simulink model "ElectricVehicleThermalManagementWithHeatPump_2026a_version"  (R2026a)
settings: Solver=VariableStepAuto  StopTime=3600  AbsTol=1e-3
PreLoadFcn:
  | init_nmpc
InitFcn:
  | init_nmpc
model workspace: external: MATLAB File ElectricVehicleThermalManagementWithHeatPumpParameters.m (data not in the file)
values from neighbouring files (symbols this model uses):
  battery_C1_LUT = [1913.6 12447 30609 ... (first row only)    [ElectricVehicleThermalManagementWithHeatPumpParameters.m]
  battery_capacity_LUT = [280.081 276.25 276.392]    [ElectricVehicleThermalManagementWithHeatPumpParameters.m]
  battery_cell_cp = 795    [ElectricVehicleThermalManagementWithHeatPumpParameters.m]
  battery_cell_mass = 2.5    [ElectricVehicleThermalManagementWithHeatPumpParameters.m]
  battery_Em_LUT = [3.4966 3.5057 3.5148 ... (first row only)    [ElectricVehicleThermalManagementWithHeatPumpParameters.m]
  battery_N_cells = 20    [ElectricVehicleThermalManagementWithHeatPumpParameters.m]
  battery_Qe_init = 0    [ElectricVehicleThermalManagementWithHeatPumpParameters.m]
  battery_R0_LUT = [0.0117 0.0085 0.009 ... (first row only)    [ElectricVehicleThermalManagementWithHeatPumpParameters.m]
  battery_R1_LUT = [0.0109 0.0029 0.0013 ... (first row only)    [ElectricVehicleThermalManagementWithHeatPumpParameters.m]
  battery_SOC_LUT = [0; 0.1; 0.25; 0.5; 0.75; 0.9; 1]    [ElectricVehicleThermalManagementWithHeatPumpParameters.m]
  battery_T_init = -5    [ElectricVehicleThermalManagementWithHeatPumpParameters.m]
  battery_temperature_LUT = [5 20 40]    [ElectricVehicleThermalManagementWithHeatPumpParameters.m]
  cabin_duct_area = 0.04    [ElectricVehicleThermalManagementWithHeatPumpParameters.m]
  cabin_T_init = -5    [ElectricVehicleThermalManagementWithHeatPumpParameters.m]
  chiller_area_primary = 0.43982297150257105    (= 0.439822971503)    [ElectricVehicleThermalManagementWithHeatPumpParameters.m]
  chiller_N_baffles = 3    [ElectricVehicleThermalManagementWithHeatPumpParameters.m]
  chiller_N_tubes = 100    [ElectricVehicleThermalManagementWithHeatPumpParameters.m]
  chiller_tube_D = 0.0035    [ElectricVehicleThermalManagementWithHeatPumpParameters.m]
  chiller_tube_L = 0.4    [ElectricVehicleThermalManagementWithHeatPumpParameters.m]
  chiller_wall_conductivity = 240    [ElectricVehicleThermalManagementWithHeatPumpParameters.m]
  chiller_wall_thickness = 0.0001    [ElectricVehicleThermalManagementWithHeatPumpParameters.m]
  cond_evap_air_area_flow = 0.3906    [ElectricVehicleThermalManagementWithHeatPumpParameters.m]
  cond_evap_air_area_primary = 1.4834999999999998    (= 1.4835)    [ElectricVehicleThermalManagementWithHeatPumpParameters.m]
  cond_evap_W = 0.015    [ElectricVehicleThermalManagementWithHeatPumpParameters.m]
  cond_evap_wall_conductivity = 240    [ElectricVehicleThermalManagementWithHeatPumpParameters.m]
  cond_evap_wall_thickness = 0.0001    [ElectricVehicleThermalManagementWithHeatPumpParameters.m]
  coolant_channel_D = 0.0092    [ElectricVehicleThermalManagementWithHeatPumpParameters.m]
  coolant_pipe_D = 0.019    [ElectricVehicleThermalManagementWithHeatPumpParameters.m]
  coolant_T_init = -5    [ElectricVehicleThermalManagementWithHeatPumpParameters.m]
  coolant_tank_area = 0.0121    [ElectricVehicleThermalManagementWithHeatPumpParameters.m]
  coolant_tank_volume = 1.25    [ElectricVehicleThermalManagementWithHeatPumpParameters.m]
  coolant_valve_D_ratio_max = 0.95    [ElectricVehicleThermalManagementWithHeatPumpParameters.m]
  coolant_valve_D_ratio_min = 0.001    [ElectricVehicleThermalManagementWithHeatPumpParameters.m]
  coolant_valve_displacement = 0.0063    [ElectricVehicleThermalManagementWithHeatPumpParameters.m]
  coolant_valve_S_max = 0.0053    [ElectricVehicleThermalManagementWithHeatPumpParameters.m]
  evaporator_air_area_flow = 0.12    [ElectricVehicleThermalManagementWithHeatPumpParameters.m]
  evaporator_air_area_primary = 0.4323    [ElectricVehicleThermalManagementWithHeatPumpParameters.m]
  evaporator_W = 0.015    [ElectricVehicleThermalManagementWithHeatPumpParameters.m]
  evaporator_wall_conductivity = 240    [ElectricVehicleThermalManagementWithHeatPumpParameters.m]
  evaporator_wall_thickness = 0.0001    [ElectricVehicleThermalManagementWithHeatPumpParameters.m]
  expansion_valve_D_ratio_max = 0.9    [ElectricVehicleThermalManagementWithHeatPumpParameters.m]
  hex_area_primary = 0.070371675440411369    (= 0.0703716754404)    [ElectricVehicleThermalManagementWithHeatPumpParameters.m]
  hex_N_tubes = 64    [ElectricVehicleThermalManagementWithHeatPumpParameters.m]
  hex_tube_D = 0.0035    [ElectricVehicleThermalManagementWithHeatPumpParameters.m]
  hex_wall_conductivity = 240    [ElectricVehicleThermalManagementWithHeatPumpParameters.m]
  hex_wall_thickness = 0.0001    [ElectricVehicleThermalManagementWithHeatPumpParameters.m]
  inner_cond_air_area_flow = 0.1953    [ElectricVehicleThermalManagementWithHeatPumpParameters.m]
  inner_cond_air_area_primary = 0.99520000000000008    (= 0.9952)    [ElectricVehicleThermalManagementWithHeatPumpParameters.m]
  inner_cond_W = 0.02    [ElectricVehicleThermalManagementWithHeatPumpParameters.m]
  inner_cond_wall_conductivity = 240    [ElectricVehicleThermalManagementWithHeatPumpParameters.m]
  inner_cond_wall_thickness = 0.0001    [ElectricVehicleThermalManagementWithHeatPumpParameters.m]
  pump_speed_max = 1000    [ElectricVehicleThermalManagementWithHeatPumpParameters.m]
  radiator_air_area_flow = 0.097499999999999989    (= 0.0975)    [ElectricVehicleThermalManagementWithHeatPumpParameters.m]
  radiator_air_area_primary = 0.43687499999999996    (= 0.436875)    [ElectricVehicleThermalManagementWithHeatPumpParameters.m]
  radiator_W = 0.015    [ElectricVehicleThermalManagementWithHeatPumpParameters.m]
  radiator_wall_conductivity = 240    [ElectricVehicleThermalManagementWithHeatPumpParameters.m]
  radiator_wall_thickness = 0.0001    [ElectricVehicleThermalManagementWithHeatPumpParameters.m]
  refrigerant_p_init = 0.25    [ElectricVehicleThermalManagementWithHeatPumpParameters.m]
  refrigerant_pipe_D = 0.01    [ElectricVehicleThermalManagementWithHeatPumpParameters.m]
  refrigerant_valve_D_ratio_max = 0.95    [ElectricVehicleThermalManagementWithHeatPumpParameters.m]
  refrigerant_valve_displacement = 0.005    [ElectricVehicleThermalManagementWithHeatPumpParameters.m]
libraries: fl_lib x227, nesl_utility x162, SimscapeFluids_lib x30, LiBatteryElements_lib x16, slpidlib x3, SignalEditorBlockLib x1
(part 3 of 13)

== system ElectricVehicleThermalManagementWithHeatPump_2026a_version/Chiller ==
  Chiller : SimscapeFluids_lib/Heat Exchangers/Two-Phase Fluid - Thermal Liquid/Condenser Evaporator (TL-2P)  flow_arrangement=fluids.heat_exchangers.enum.FlowArrangementTL2P.Cross  cross_flow_arrangement=fluids.heat_exchangers.enum.CrossFlowArrangementTL2P.UnmixedMixed  R_wall=chiller_wall_thickness / chiller_area_primary / chiller_wall_conductivity K/W  wall_thermal_mass=false  mass_wall=1 kg  cp_wall=490 J/(K*kg)  area_A1=pi * coolant_pipe_D^2 / 4 m^2  area_B1=pi * coolant_pipe_D^2 / 4 m^2  area_A2=pi * refrigerant_pipe_D^2 / 4 m^2  area_B2=pi * refrigerant_pipe_D^2 / 4 m^2  flow_geometry_TL=fluids.heat_exchangers.enum.FlowGeometryTL.AcrossTubeBank  tube_num_TL=1  tube_length_TL=5 m  tube_cross_section_TL=fluids.heat_exchangers.enum.TubeCrossSection.Circular  tube_diameter_TL=0.1 m  tube_width_TL=0.1 m  tube_height_TL=0.1 m  tube_inner_diameter_TL=0.05 m  tube_outer_diameter_TL=0.1 m  tube_flow_area_TL=0.01 m^2  tube_wetted_perimeter_TL=0.4 m  tube_heat_perimeter_TL=0.4 m  tube_pressure_loss_spec_TL=fluids.heat_exchangers.enum.TubePressureLossSpec.Haaland  tube_loss_coeff_TL=10  tube_local_pressure_loss_spec_TL=fluids.heat_exchangers.enum.LocalLossSpec.AggregateLength  tube_length_add_TL=0.1 m  tube_local_loss_coefficient_TL=0.1  tube_roughness_pressure_TL=15e-6 m  tube_Re_lam_pressure_TL=2000  tube_Re_tur_pressure_TL=4000  tube_shape_factor_generic_TL=64  tube_heat_coeff_spec_TL=fluids.heat_exchangers.enum.TubeHeatCoeffSpec.Gneilinski  tube_colburn_coeff_TL=[.023, .8, .33]  tube_roughness_heat_TL=15e-6 m  tube_Re_lam_heat_TL=2000  tube_Re_tur_heat_TL=4000  tube_Nu_lam_generic_TL=3.66  bank_arrangement_TL=fluids.heat_exchangers.enum.BankArrangement.Staggered  bank_num_rows_TL=sqrt(chiller_N_tubes) * (chiller_N_baffles + 1)  bank_tubes_per_row_TL=sqrt(chiller_N_tubes)  bank_width_TL=chiller_tube_L / (chiller_N_baffles + 1) m  bank_tube_diameter_TL=chiller_tube_D m  bank_longitudinal_pitch_TL=2 * chiller_tube_D m  bank_transverse_pitch_TL=2 * chiller_tube_D m  bank_pressure_loss_spec_TL=fluids.heat_exchangers.enum.BankPressureLossSpec.Martin  bank_euler_TL=10  bank_heat_coeff_spec_TL=fluids.heat_exchangers.enum.BankHeatCoeffSpec.Martin  bank_colburn_coeff_TL=[.27, .63, .36]  generic_flow_area_TL=0.01 m^2  generic_heat_area_TL=2 m^2  generic_volume_TL=0.05 m^3  generic_loss_coeff_TL=10  generic_colburn_coeff_TL=[.023, .8, .33]  fouling_factor_TL=0.1 m^2*K/kW  fin_area_TL=chiller_area_baffles m^2  fin_efficiency_TL=0.5  p_init_TL=coolant_p_init MPa  T_init_TL=coolant_T_init degC  tube_num_2P=chiller_N_tubes  tube_length_2P=chiller_tube_L m  tube_cross_section_2P=fluids.heat_exchangers.enum.TubeCrossSection.Circular  tube_diameter_2P=chiller_tube_D m  tube_width_2P=0.1 m  tube_height_2P=0.1 m  tube_inner_diameter_2P=0.05 m  tube_outer_diameter_2P=0.1 m  tube_flow_area_2P=0.01 m^2  tube_wetted_perimeter_2P=0.4 m  tube_heat_perimeter_2P=0.4 m  tube_pressure_loss_spec_2P=fluids.heat_exchangers.enum.TubePressureLossSpec2P.Haaland  tube_loss_coeff_2P=10  tube_local_pressure_loss_spec_2P=fluids.heat_exchangers.enum.LocalLossSpec.AggregateLength  tube_length_add_2P=chiller_tube_Leq m  tube_local_loss_coefficient_2P=0.1  tube_roughness_pressure_2P=15e-6 m  tube_Re_lam_pressure_2P=2000  tube_Re_tur_pressure_2P=4000  tube_shape_factor_generic_2P=64  tube_heat_coeff_spec_2P=fluids.heat_exchangers.enum.TubeHeatCoeffSpec2P.GneilinskiCavalliniZecchin  tube_colburn_coeff_liq_2P=[.023, .8, .33]  tube_colburn_coeff_mix_2P=[.05, .8, .33]  tube_colburn_coeff_vap_2P=[.023, .8, .33]  tube_roughness_heat_2P=15e-6 m  tube_Re_lam_heat_2P=2000  tube_Re_tur_heat_2P=4000  tube_Nu_lam_generic_2P=3.66  fouling_factor_2P=0.1 m^2*K/kW  fin_area_2P=0 m^2  fin_efficiency_2P=0  energy_spec_2P=foundation.enum.energy_spec.void_fraction  p_init_2P=refrigerant_p_init MPa  T_init_2P=293.15 K  x_init_2P=0.5  alpha_init_2P=refrigerant_alpha_init  h_init_2P=1500 kJ/kg  u_init_2P=1500 kJ/kg
  Flow Resistance (2P) : fl_lib/Two-Phase Fluid/Elements/Flow Resistance (2P)  delta_p_nominal=1e-4 MPa  mdot_nominal=0.01 kg/s  v_nominal=0 m^3/kg  area=pi * refrigerant_pipe_D^2 / 4 m^2  laminar_fraction=1e-3
  PS-Simulink Converter : nesl_utility/PS-Simulink Converter  PhysicalDomain=network_engine_domain  SubClassName=ps_output  LeftPortType=input  RightPortType=output  PseudoPeriodic=off  Frequencies=[]  VectorFormat=inherit  Unit=inherit  AffineConversion=off
  PS-Simulink Converter1 : nesl_utility/PS-Simulink Converter  PhysicalDomain=network_engine_domain  SubClassName=ps_output  LeftPortType=input  RightPortType=output  PseudoPeriodic=off  Frequencies=[]  VectorFormat=inherit  Unit=inherit  AffineConversion=off
  Pressure & Temperature Sensor (TL) : fl_lib/Thermal Liquid/Sensors/Pressure & Temperature Sensor (TL)  reference=foundation.enum.MeasurementReference.absolute  pressure=true  pressure_spec=foundation.enum.PressureMeasementSpec.Absolute  temperature=true
  Pressure & Temperature Sensor (TL)1 : fl_lib/Thermal Liquid/Sensors/Pressure & Temperature Sensor (TL)  reference=foundation.enum.MeasurementReference.absolute  pressure=true  pressure_spec=foundation.enum.PressureMeasementSpec.Absolute  temperature=true
  SR10 : Subsystem
  SR9 : Subsystem
  To Workspace : ToWorkspace  VariableName=clntChilTemp_in  SampleTime=-1
  To Workspace1 : ToWorkspace  VariableName=clntChilTemp_out  SampleTime=-1
  C : PMIOPort  Side=Left
  A : PMIOPort  Port=2  Side=Left
  D : PMIOPort  Port=3  Side=Right
  B : PMIOPort  Port=4  Side=Right
  wires:
  PS-Simulink Converter/1 -> To Workspace/1
  PS-Simulink Converter1/1 -> To Workspace1/1
  connections:
  SR10/LConn1 -- Chiller/RConn2
  SR10/RConn1 -- Flow Resistance (2P)/LConn1
  B/RConn1 -- Flow Resistance (2P)/RConn1
  SR9/RConn1 -- Chiller/RConn1
  Chiller/LConn2 -- Pressure & Temperature Sensor (TL)1/LConn1 -- D/RConn1
  Chiller/LConn1 -- Pressure & Temperature Sensor (TL)/LConn1 -- C/RConn1
  SR9/LConn1 -- A/RConn1
  PS-Simulink Converter/LConn1 -- Pressure & Temperature Sensor (TL)/RConn2
  PS-Simulink Converter1/LConn1 -- Pressure & Temperature Sensor (TL)1/RConn2

== system ElectricVehicleThermalManagementWithHeatPump_2026a_version/Chiller Expansion Valve ==
  Chiller Expansion Valve : SimscapeFluids_lib/Two-Phase Fluid/Valves & Orifices/Orifice (2P)  orifice_type=foundation.enum.constant_variable.variable  constant_liquid_orifice_parameterization=fluids.two_phase_fluid.valves_orifices.enum.LiquidConstantOrificeParameterization.Area  variable_liquid_orifice_parameterization=fluids.two_phase_fluid.valves_orifices.enum.LiquidOrificeParameterization.LinearArea  mdot_nominal_constant=0.1 kg/s  delta_p_nominal_constant=0.001 MPa  orifice_area_constant=1e-4 m^2  S_min=0 m  del_S=refrigerant_valve_displacement m  open_orientation=fluids.two_phase_fluid.valves_orifices.enum.OrificeOrientation.Positive  mdot_nominal_max=0.1 kg/s  delta_p_nominal_max=0.001 MPa  orifice_area_max=pi * (expansion_valve_D_ratio_max*refrigerant_pipe_D)^2 / 4 m^2  S_TLU=[0, .002, .004, .007, .017] m  orifice_area_TLU=[1e-10, 2e-05, 4e-05, 6e-05, 8e-05, .0001] m^2  energy_spec=foundation.enum.energy_spec.temperature  p_inlet=0.101325 MPa  T_inlet=293.15 K  x_inlet=0  alpha_inlet=0  h_inlet=400 kJ/kg  u_inlet=400 kJ/kg  Cd=0.7  pressure_recovery=true  leakage_fraction=1e-6  smoothing_factor=0.01  B_lam=0.999  tau_x=0.1 s  area=pi * refrigerant_pipe_D^2 / 4 m^2  vapor_orifice_parameterization=fluids.two_phase_fluid.valves_orifices.enum.VaporOrificeParameterization.Cv  opening_characteristic=fluids.two_phase_fluid.valves_orifices.enum.OpeningCharacteristics.Linear  Cv_constant=4  Cv_max=4  S_Cv_TLU=[0, .003, .006, .009, .012, .015] m  Cv_TLU=[1e-06, .8, 1.6, 2.4, 3.2, 4]  xT_Cv=0.7  Kv_constant=3.6  Kv_max=3.6  S_Kv_TLU=[0, .003, .006, .009, .012, .015] m  Kv_TLU=[1e-06, .72, 1.44, 2.16, 2.88, 3.6]  xT_Kv=0.7  S_orifice_area_TLU=[0, .003, .006, .009, .012, .015] m
  Display : Display
  Max Valve Displacement [m] : Gain  Gain=refrigerant_valve_displacement
  Scope : Scope
      settings: ActiveDisplayYMinimum=-0.003  ActiveDisplayYMaximum=0.027  DataLoggingVariableName=ScopeData3
  Scope1 : Scope
      settings: ActiveDisplayYMinimum=-0.003  ActiveDisplayYMaximum=0.027  DataLoggingVariableName=ScopeData4
  Scope2 : Scope
      settings: ActiveDisplayYMinimum=-1E-5  ActiveDisplayYMaximum=0.00014  DataLoggingVariableName=ScopeData5
  Simulink-PS Converter : nesl_utility/Simulink-PS Converter  PhysicalDomain=network_engine_domain  SubClassName=ps_input  LeftPortType=input  RightPortType=output  PseudoPeriodic=off  Frequencies=[]  NoiseDistribution=none  NoiseParameters=[]  Unit=m  AffineConversion=off  FilteringAndDerivatives=provide  SimscapeFilterOrder=1  InputFilterTimeConstant=0.001  UdotUserProvided=0
  Transfer Fcn : TransferFcn  Denominator=[1 1]
  A : PMIOPort  Side=Left
  B : PMIOPort  Port=2  Side=Right
  wires:
  Max Valve Displacement [m]/1 -> Display/1, Scope2/1, Simulink-PS Converter/1
  [cmd_exv_chiller] -> Scope1/1, Transfer Fcn/1
  Transfer Fcn/1 -> Scope/1, Max Valve Displacement [m]/1
  connections:
  Chiller Expansion Valve/RConn1 -- B/RConn1
  Chiller Expansion Valve/LConn1 -- A/RConn1
  Chiller Expansion Valve/LConn2 -- Simulink-PS Converter/RConn1

== system ElectricVehicleThermalManagementWithHeatPump_2026a_version/Chiller Evaporator Bypass Valve ==
  Bias : Bias  Bias=-1  SaturateOnIntegerOverflow=off
  Gain : Gain  Gain=2
  Max Valve Displacement [m] : Gain  Gain=refrigerant_valve_displacement
  Orifice AB : SimscapeFluids_lib/Two-Phase Fluid/Valves & Orifices/Orifice (2P)  orifice_type=foundation.enum.constant_variable.variable  constant_liquid_orifice_parameterization=fluids.two_phase_fluid.valves_orifices.enum.LiquidConstantOrificeParameterization.Area  variable_liquid_orifice_parameterization=fluids.two_phase_fluid.valves_orifices.enum.LiquidOrificeParameterization.LinearArea  mdot_nominal_constant=0.1 kg/s  delta_p_nominal_constant=0.001 MPa  orifice_area_constant=1e-4 m^2  S_min=-0.8*refrigerant_valve_displacement m  del_S=refrigerant_valve_displacement m  open_orientation=fluids.two_phase_fluid.valves_orifices.enum.OrificeOrientation.Positive  mdot_nominal_max=0.1 kg/s  delta_p_nominal_max=0.001 MPa  orifice_area_max=pi * (refrigerant_valve_D_ratio_max*refrigerant_pipe_D)^2 / 4 m^2  S_TLU=[0, .002, .004, .007, .017] m  orifice_area_TLU=[1e-10, 2e-05, 4e-05, 6e-05, 8e-05, .0001] m^2  energy_spec=foundation.enum.energy_spec.temperature  p_inlet=0.101325 MPa  T_inlet=293.15 K  x_inlet=0  alpha_inlet=0  h_inlet=400 kJ/kg  u_inlet=400 kJ/kg  Cd=0.7  pressure_recovery=true  leakage_fraction=1e-6  smoothing_factor=0.01  B_lam=0.999  tau_x=0.1 s  area=pi * refrigerant_pipe_D^2 / 4 m^2  vapor_orifice_parameterization=fluids.two_phase_fluid.valves_orifices.enum.VaporOrificeParameterization.Cv  opening_characteristic=fluids.two_phase_fluid.valves_orifices.enum.OpeningCharacteristics.Linear  Cv_constant=4  Cv_max=4  S_Cv_TLU=[0, .003, .006, .009, .012, .015] m  Cv_TLU=[1e-06, .8, 1.6, 2.4, 3.2, 4]  xT_Cv=0.7  Kv_constant=3.6  Kv_max=3.6  S_Kv_TLU=[0, .003, .006, .009, .012, .015] m  Kv_TLU=[1e-06, .72, 1.44, 2.16, 2.88, 3.6]  xT_Kv=0.7  S_orifice_area_TLU=[0, .003, .006, .009, .012, .015] m
  Orifice AC : SimscapeFluids_lib/Two-Phase Fluid/Valves & Orifices/Orifice (2P)  orifice_type=foundation.enum.constant_variable.variable  constant_liquid_orifice_parameterization=fluids.two_phase_fluid.valves_orifices.enum.LiquidConstantOrificeParameterization.Area  variable_liquid_orifice_parameterization=fluids.two_phase_fluid.valves_orifices.enum.LiquidOrificeParameterization.LinearArea  mdot_nominal_constant=0.1 kg/s  delta_p_nominal_constant=0.001 MPa  orifice_area_constant=1e-4 m^2  S_min=0.8*refrigerant_valve_displacement m  del_S=refrigerant_valve_displacement m  open_orientation=fluids.two_phase_fluid.valves_orifices.enum.OrificeOrientation.Negative  mdot_nominal_max=0.1 kg/s  delta_p_nominal_max=0.001 MPa  orifice_area_max=pi * (refrigerant_valve_D_ratio_max*refrigerant_pipe_D)^2 / 4 m^2  S_TLU=[0, .002, .004, .007, .017] m  orifice_area_TLU=[1e-10, 2e-05, 4e-05, 6e-05, 8e-05, .0001] m^2  energy_spec=foundation.enum.energy_spec.temperature  p_inlet=0.101325 MPa  T_inlet=293.15 K  x_inlet=0  alpha_inlet=0  h_inlet=400 kJ/kg  u_inlet=400 kJ/kg  Cd=0.7  pressure_recovery=true  leakage_fraction=1e-6  smoothing_factor=0.01  B_lam=0.999  tau_x=0.1 s  area=pi * refrigerant_pipe_D^2 / 4 m^2  vapor_orifice_parameterization=fluids.two_phase_fluid.valves_orifices.enum.VaporOrificeParameterization.Cv  opening_characteristic=fluids.two_phase_fluid.valves_orifices.enum.OpeningCharacteristics.Linear  Cv_constant=4  Cv_max=4  S_Cv_TLU=[0, .003, .006, .009, .012, .015] m  Cv_TLU=[1e-06, .8, 1.6, 2.4, 3.2, 4]  xT_Cv=0.7  Kv_constant=3.6  Kv_max=3.6  S_Kv_TLU=[0, .003, .006, .009, .012, .015] m  Kv_TLU=[1e-06, .72, 1.44, 2.16, 2.88, 3.6]  xT_Kv=0.7  S_orifice_area_TLU=[0, .003, .006, .009, .012, .015] m
  Scope : Scope
      settings: ActiveDisplayYMinimum=-1  ActiveDisplayYMaximum=1  DataLoggingVariableName=ScopeData2
  Simulink-PS Converter : nesl_utility/Simulink-PS Converter  PhysicalDomain=network_engine_domain  SubClassName=ps_input  LeftPortType=input  RightPortType=output  PseudoPeriodic=off  Frequencies=[]  NoiseDistribution=none  NoiseParameters=[]  Unit=m  AffineConversion=off  FilteringAndDerivatives=provide  SimscapeFilterOrder=1  InputFilterTimeConstant=0.001  UdotUserProvided=0
  Transfer Fcn : TransferFcn  Denominator=[1 1]
  C : PMIOPort  Side=Left
  A : PMIOPort  Port=2  Side=Right
  B : PMIOPort  Port=3  Side=Right
  wires:
  Transfer Fcn/1 -> Gain/1
  Bias/1 -> Max Valve Displacement [m]/1
  [cmd_refrig_bypass] -> Scope/1, Transfer Fcn/1
  Max Valve Displacement [m]/1 -> Simulink-PS Converter/1
  Gain/1 -> Bias/1
  connections:
  A/RConn1 -- Orifice AB/LConn1 -- Orifice AC/LConn1
  Orifice AC/RConn1 -- C/RConn1
  Orifice AB/RConn1 -- B/RConn1
  Simulink-PS Converter/RConn1 -- Orifice AB/LConn2 -- Orifice AC/LConn2

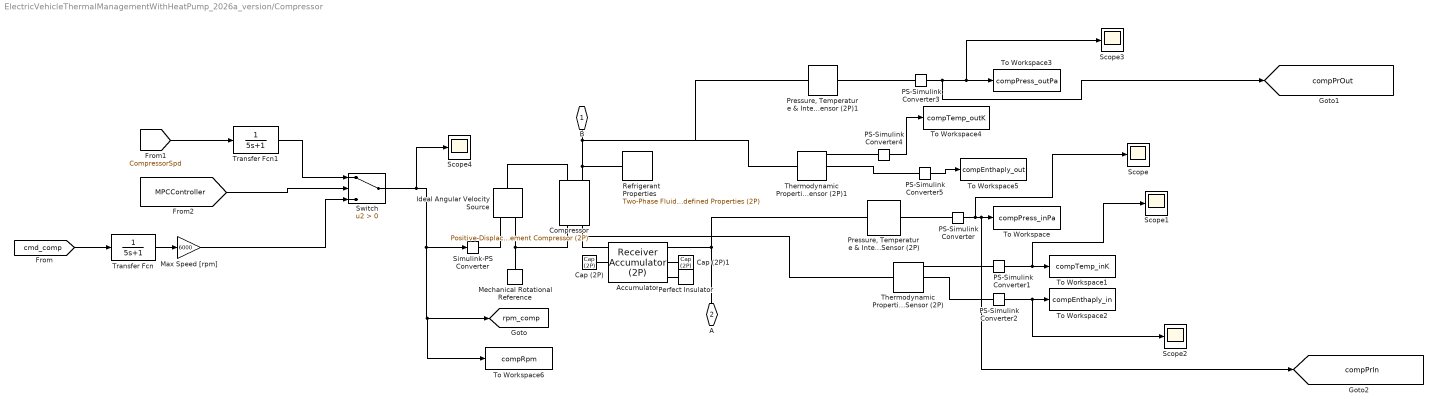
== system ElectricVehicleThermalManagementWithHeatPump_2026a_version/Compressor ==
  Accumulator : SimscapeFluids_lib/Two-Phase Fluid/Tanks & Accumulators/Receiver Accumulator (2P)  volume=4 l  tank_area=0.5 m^2  area_AV=pi * refrigerant_pipe_D^2 / 4 m^2  area_BV=pi * refrigerant_pipe_D^2 / 4 m^2  area_AL=pi * refrigerant_pipe_D^2 / 4 m^2  area_BL=pi * refrigerant_pipe_D^2 / 4 m^2  V_frac_liq_error=simscape.enum.assert.action.none  V_frac_liq_min=0.05  V_frac_liq_max=0.95  V_frac_smooth=0.05  p_crit_error=simscape.enum.assert.action.error  hc_vap=20 W/(K*m^2)  hc_liq=100 W/(K*m^2)  p_init=refrigerant_p_init MPa  fraction_spec=fluids.two_phase_fluid.tanks_accumulators.enum.LiquidFractionSpec.Volume  M_frac_liq_init=0.5  V_frac_liq_init=0.1  saturated_init=true  energy_spec=fluids.two_phase_fluid.tanks_accumulators.enum.EnergySpec.SubcoolingSuperheating  delta_T_sub_init=5 deltaK  delta_T_sup_init=5 deltaK  T_liq_init=368.15 K  T_vap_init=378.15 K  h_liq_init=400 kJ/kg  h_vap_init=2700 kJ/kg  u_liq_init=400 kJ/kg  u_vap_init=2700 kJ/kg  tau_vap_cond=0.1 s
  Cap (2P) : fl_lib/Two-Phase Fluid/Elements/Cap (2P)  p_specify=off  p_priority=None  p=0.101325 MPa  p_nominal_specify=off  p_nominal_value=1  p_nominal_unit=MPa  u_specify=off  u_priority=None  u=1500 kJ/kg  u_nominal_specify=off  u_nominal_value=1  u_nominal_unit=kJ/kg
  Cap (2P)1 : fl_lib/Two-Phase Fluid/Elements/Cap (2P)  p_specify=off  p_priority=None  p=0.101325 MPa  p_nominal_specify=off  p_nominal_value=1  p_nominal_unit=MPa  u_specify=off  u_priority=None  u=1500 kJ/kg  u_nominal_specify=off  u_nominal_value=1  u_nominal_unit=kJ/kg
  Compressor : SimscapeFluids_lib/Two-Phase Fluid/Fluid Machines/Positive-Displacement Compressor (2P)  dispSpec=fluids.two_phase_fluid.fluid_machines.enum.DisplacementSpecification.Displacement  v_disp=compressor_displacement cm^3/rev  mdot_nom=0.01 kg/s  omega_nom=1000 rpm  efficiencySpec=fluids.two_phase_fluid.fluid_machines.enum.VolumetricEfficiencyParameterization.Analytical  thermodynamicModelSpec=fluids.two_phase_fluid.fluid_machines.enum.ThermodynamicModel.Isentropic  n=1.2  eta_isen=0.65  eta_isen_TLU=[.95, .9, .85, .8, .75; .925, .875, .825, .775, .725; .875, .825, .775, .725, .675; .75, .7, .65, .6, .55]  eta_vol_nom=0.9  pr_TLU=[2, 4, 6, 8]  omega_TLU=[800, 1500, 2800, 3300, 4000] rpm  eta_vol_TLU=[.95, .9, .85, .8, .75; .925, .875, .825, .775, .725; .875, .825, .775, .725, .675; .75, .7, .65, .6, .55]  nominalSpec=fluids.two_phase_fluid.fluid_machines.enum.NominalConditionsSpecification.Pressure  pr_nom=4.6  p_in_nom=0.3 MPa  T_in_nom=11 degC  T_evap_nom=373.15 K  T_cond_nom=398.15 K  delta_T_nom=10 deltaK  mechanical_efficiency=0.95  area_A=pi * refrigerant_pipe_D^2 / 4 m^2  area_B=pi * refrigerant_pipe_D^2 / 4 m^2  VaporCheck=simscape.enum.assert.action.none
  Ideal Angular Velocity Source : fl_lib/Mechanical/Mechanical Sources/Ideal Angular Velocity Source
  Max Speed [rpm] : Gain  Gain=6000
  Mechanical Rotational Reference : fl_lib/Mechanical/Rotational Elements/Mechanical Rotational Reference
  PS-Simulink Converter{,1..5} (6 alike) : nesl_utility/PS-Simulink Converter  PhysicalDomain=network_engine_domain  SubClassName=ps_output  LeftPortType=input  RightPortType=output  PseudoPeriodic=off  Frequencies=[]  VectorFormat=inherit  Unit=inherit  AffineConversion=off
  Perfect Insulator : fl_lib/Thermal/Thermal Elements/Perfect Insulator  T_specify=off  T_priority=None  T=293.15 K  T_nominal_specify=off  T_nominal_value=1  T_nominal_unit=K
  "Pressure, Temperature & Internal Energy Sensor (2P)" : fl_lib/Two-Phase Fluid/Sensors/Pressure, Temperature & Internal Energy Sensor (2P)  reference=foundation.enum.MeasurementReference.absolute  pressure=true  pressure_spec=foundation.enum.PressureMeasementSpec.Absolute  temperature=false  internal_energy=false
  "Pressure, Temperature & Internal Energy Sensor (2P)1" : fl_lib/Two-Phase Fluid/Sensors/Pressure, Temperature & Internal Energy Sensor (2P)  reference=foundation.enum.MeasurementReference.absolute  pressure=true  pressure_spec=foundation.enum.PressureMeasementSpec.Absolute  temperature=false  internal_energy=false
  Refrigerant Properties : SimscapeFluids_lib/Two-Phase Fluid/Utilities/Two-Phase Fluid Predefined Properties (2P)  fluid=fluids.two_phase_fluid.utilities.enum.Fluid.R134a  p_atm=0.101325 MPa  properties_range_check=simscape.enum.assert.action.error  q_rev=0.01 Pa
  Scope{,1..4} (5 alike) : Scope
      Scope settings: ActiveDisplayYMinimum=0.05986  ActiveDisplayYMaximum=0.28314  DataLoggingVariableName=ScopeData10
      Scope1 settings: ActiveDisplayYMinimum=241.45357  ActiveDisplayYMaximum=273.1745  DataLoggingVariableName=ScopeData11
      Scope2 settings: ActiveDisplayYMinimum=334.35031  ActiveDisplayYMaximum=407.78163  DataLoggingVariableName=ScopeData12
      Scope3 settings: ActiveDisplayYMinimum=-0.28873  ActiveDisplayYMaximum=4.5986
      Scope4 settings: ActiveDisplayYMinimum=-746.11242  ActiveDisplayYMaximum=6715.0118  DataLoggingVariableName=ScopeData4
  Simulink-PS Converter : nesl_utility/Simulink-PS Converter  PhysicalDomain=network_engine_domain  SubClassName=ps_input  LeftPortType=input  RightPortType=output  PseudoPeriodic=off  Frequencies=[]  NoiseDistribution=none  NoiseParameters=[]  Unit=rpm  AffineConversion=off  FilteringAndDerivatives=provide  SimscapeFilterOrder=1  InputFilterTimeConstant=0.001  UdotUserProvided=0
  Switch : Switch  Criteria=u2 > Threshold  SaturateOnIntegerOverflow=off  InputSameDT=off
  Thermodynamic Properties Sensor (2P) : fl_lib/Two-Phase Fluid/Sensors/Thermodynamic Properties Sensor (2P)  temperature=true  enthalpy=true  density=true  specific_volume=false  entropy=false
  Thermodynamic Properties Sensor (2P)1 : fl_lib/Two-Phase Fluid/Sensors/Thermodynamic Properties Sensor (2P)  temperature=true  enthalpy=true  density=true  specific_volume=false  entropy=false
  To Workspace : ToWorkspace  VariableName=compPress_inPa  SampleTime=-1
  To Workspace1 : ToWorkspace  VariableName=compTemp_inK  SampleTime=-1
  To Workspace2 : ToWorkspace  VariableName=compEnthaply_in  SampleTime=-1
  To Workspace3 : ToWorkspace  VariableName=compPress_outPa  SampleTime=-1
  To Workspace4 : ToWorkspace  VariableName=compTemp_outK  SampleTime=-1
  To Workspace5 : ToWorkspace  VariableName=compEnthaply_out  SampleTime=-1
  To Workspace6 : ToWorkspace  VariableName=compRpm  SampleTime=-1
  Transfer Fcn : TransferFcn  Denominator=[5 1]
  Transfer Fcn1 : TransferFcn  Denominator=[5 1]
  B : PMIOPort  Side=Left
  A : PMIOPort  Port=2  Side=Right
  tag scope: compPrIn=global, compPrOut=global, rpm_comp=global
  wires:
  Transfer Fcn/1 -> Max Speed [rpm]/1
  [cmd_comp] -> Transfer Fcn/1
  Max Speed [rpm]/1 -> Switch/3
  PS-Simulink Converter/1 -> Scope/1, [compPrIn], To Workspace/1
  PS-Simulink Converter1/1 -> Scope1/1, To Workspace1/1
  PS-Simulink Converter2/1 -> Scope2/1, To Workspace2/1
  PS-Simulink Converter3/1 -> [compPrOut], Scope3/1, To Workspace3/1
  PS-Simulink Converter4/1 -> To Workspace4/1
  PS-Simulink Converter5/1 -> To Workspace5/1
  [MPCController] -> Switch/2
  [CompressorSpd] -> Transfer Fcn1/1
  Switch/1 -> To Workspace6/1, [rpm_comp], Simulink-PS Converter/1, Scope4/1
  Transfer Fcn1/1 -> Switch/1
  connections:
  Simulink-PS Converter/RConn1 -- Ideal Angular Velocity Source/RConn1
  B/RConn1 -- "Pressure, Temperature & Internal Energy Sensor (2P)1"/LConn1 -- Thermodynamic Properties Sensor (2P)1/LConn1 -- Refrigerant Properties/RConn1 -- Compressor/RConn1
  Ideal Angular Velocity Source/LConn1 -- Compressor/RConn2
  Compressor/LConn2 -- Ideal Angular Velocity Source/RConn2 -- Mechanical Rotational Reference/LConn1
  A/RConn1 -- "Pressure, Temperature & Internal Energy Sensor (2P)"/LConn1 -- Accumulator/LConn1
  Accumulator/RConn1 -- Thermodynamic Properties Sensor (2P)/LConn1 -- Compressor/LConn1
  Cap (2P)/LConn1 -- Accumulator/RConn2
  Cap (2P)1/LConn1 -- Accumulator/LConn2
  Perfect Insulator/LConn1 -- Accumulator/LConn3
  PS-Simulink Converter/LConn1 -- "Pressure, Temperature & Internal Energy Sensor (2P)"/RConn1
  PS-Simulink Converter1/LConn1 -- Thermodynamic Properties Sensor (2P)/RConn1
  PS-Simulink Converter2/LConn1 -- Thermodynamic Properties Sensor (2P)/RConn2
  PS-Simulink Converter3/LConn1 -- "Pressure, Temperature & Internal Energy Sensor (2P)1"/RConn1
  PS-Simulink Converter4/LConn1 -- Thermodynamic Properties Sensor (2P)1/RConn1
  PS-Simulink Converter5/LConn1 -- Thermodynamic Properties Sensor (2P)1/RConn2
